simulink library "lindiCopter_lib"  (R2018b)
settings: Solver=VariableStepAuto  StartTime=0.0  StopTime=10.0  RelTol=1e-3
undefined symbols (not defined in the file or in its folder): lindi
libraries: filters_lib x5, indi_lib x4, cntrlPosNdi_lib x2, traj_lib x1, axes_transformation_lib x1, cntrlAttiRedIndi_lib x1
settings Model: Creator=Ybeyer  LastModifiedBy=yannic
settings SFSimCC: SimUseLocalCustomCode=off
settings RTWCC: RTWUseLocalCustomCode=off
settings CodeAppCC: StateflowObjectComments=on

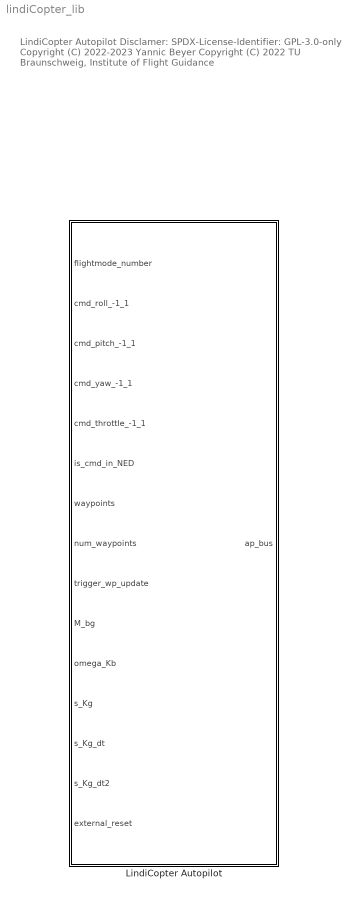
== system lindiCopter_lib ==
  note: LindiCopter Autopilot
      |
      | Disclamer:
      | SPDX-License-Identifier: GPL-3.0-only
      |
      | Copyright (C) 2022-2023 Yannic Beyer
      | Copyright (C) 2022 TU Braunschweig, Institute of Flight Guidance
  LindiCopter Autopilot : Subsystem  mask{ap=lindi}
      mask prompts: ap "LinidCopter parameters struct, see lindiCopter_params_default"
      mask init:
      | lindiCopterStateLogicBus();
      mask Help: web('hhttps://github.com/iff-gsc/LADAC/tree/main/control/autopilots/LindiCopter/README.md','-browser')
      mask DialogControl DescGroupVar Prompt: LindiCopter Autopilot
      mask DialogControl Control4 Prompt: The documentation of this block can be found here:
      mask DialogControl Control5 Prompt: README
      mask DialogControl Control5 Callback: web('https://github.com/iff-gsc/LADAC/blob/main/control/autopilots/LindiCopter/README.md','-browser')

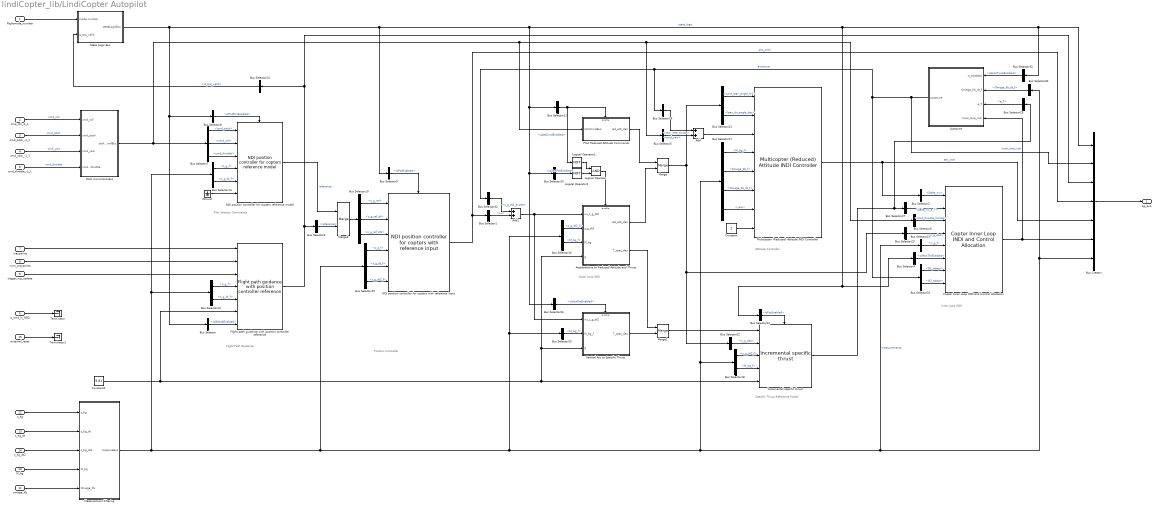
== system lindiCopter_lib/LindiCopter Autopilot ==
  note: Position Controller
  note: Flight Path Guidance
  note: Pilot Velocity Commands
  note: Outer Loop INDI
  note: Specific Thrust
      | Reference Model
  note: Attitude Controller
  note: Inner Loop INDI
  flightmode_number : Inport  SampleTime=ap.ts
  cmd_roll_-1_1 : Inport  Port=2  SampleTime=ap.ts
  cmd_pitch_-1_1 : Inport  Port=3  SampleTime=ap.ts
  cmd_yaw_-1_1 : Inport  Port=4  SampleTime=ap.ts
  cmd_throttle_-1_1 : Inport  Port=5  SampleTime=ap.ts
  is_cmd_in_NED : Inport  Port=6  SampleTime=ap.ts
  waypoints : Inport  Port=7  SampleTime=ap.ts
  num_waypoints : Inport  Port=8  SampleTime=ap.ts
  trigger_wp_update : Inport  Port=9  SampleTime=ap.ts
  M_bg : Inport  Port=10  SampleTime=ap.ts
  omega_Kb : Inport  Port=11  SampleTime=ap.ts
  s_Kg : Inport  Port=12  SampleTime=ap.ts
  s_Kg_dt : Inport  Port=13  SampleTime=ap.ts
  s_Kg_dt2 : Inport  Port=14  SampleTime=ap.ts
  external_reset : Inport  Port=15  SampleTime=ap.ts
  Accelerations to Reduced Attitude and Thrust : Subsystem
  Add : Sum
  Add1 : Sum
  Autotune : Subsystem
  Bus Creator : BusCreator  Inputs=7
  Bus Selector : BusSelector  OutputSignals=isGdnceEnabled
  Bus Selector1 : BusSelector  OutputSignals=pseudo_control.nu
  Bus Selector10 : BusSelector  OutputSignals=s_g_ref,s_g_ref_dt,s_g_ref_dt2
  Bus Selector11 : BusSelector  OutputSignals=isAttiCmdEnabled
  Bus Selector12 : BusSelector  OutputSignals=isPscEnabled
  Bus Selector13 : BusSelector  OutputSignals=s_g_f,s_g_dt_f
  Bus Selector14 : BusSelector  OutputSignals=s_g_f,s_g_dt_f
  Bus Selector15 : BusSelector  OutputSignals=s_g_f,s_g_dt_f,s_g_dt2_f
  Bus Selector16 : BusSelector  OutputSignals=s_g_dt2_f,M_bg_f
  Bus Selector17 : BusSelector  OutputSignals=M_bg_f,Omega_Kb_f,Omega_Kb_dt_f,yaw
  Bus Selector18 : BusSelector  OutputSignals=s_g_dt2_f,M_bg_f
  Bus Selector19 : BusSelector  OutputSignals=n_g_f
  Bus Selector2 : BusSelector  OutputSignals=pseudo_control.Delta_ny
  Bus Selector20 : BusSelector  OutputSignals=isVertPscEnabled
  Bus Selector21 : BusSelector  OutputSignals=cmd_lean_angle_0-1,lean_dir_angle_des
  Bus Selector22 : BusSelector  OutputSignals=n_g_des
  Bus Selector23 : BusSelector  OutputSignals=n_g_des
  Bus Selector24 : BusSelector  OutputSignals=is_traj_valid
  Bus Selector25 : BusSelector  OutputSignals=M_bg_f
  Bus Selector26 : BusSelector  OutputSignals=isVertPscEnabled
  Bus Selector27 : BusSelector  OutputSignals=Delta_nu_a_T
  Bus Selector28 : BusSelector  OutputSignals=excite.yaw_rate_excite
  Bus Selector29 : BusSelector  OutputSignals=a_T
  Bus Selector3 : BusSelector  OutputSignals=reference
  Bus Selector30 : BusSelector  OutputSignals=Omega_Kb_dt_f
  Bus Selector31 : BusSelector  OutputSignals=G1_adapt,G2_adapt
  Bus Selector32 : BusSelector  OutputSignals=excite.s_g_dt2_excite
  Bus Selector33 : BusSelector  OutputSignals=isAutoTuneEnabled
  Bus Selector4 : BusSelector  OutputSignals=isManThrEnabled
  Bus Selector5 : BusSelector  OutputSignals=cmd_yaw
  Bus Selector6 : BusSelector  OutputSignals=cmd_throttle_limited
  Bus Selector7 : BusSelector  OutputSignals=cmd_pitch,cmd_roll,cmd_throttle
  Bus Selector8 : BusSelector  OutputSignals=isPosRmEnabled
  Bus Selector9 : BusSelector  OutputSignals=isPscEnabled
  Constant : Constant
  Constant2 : Constant  Value=9.81
  Copter Inner Loop INDI and Control Allocation : indi_lib/Copter Inner Loop INDI and Control Allocation  cep=ap.cep  ceb=ap.ceb  ca=ap.ca  mtc=ap.mtc  sflt=ap.sflt  ts=ap.ts  is_ce_extern=on
      settings: SourceProductName=LADAC
  Flight path guidance with position controller reference : traj_lib/Flight path guidance with position controller reference  traj_params=ap.traj  T_inner_loop=2./ap.atc.rm.leanfreq + ap.mtc + 2./ap.sflt.omega
      settings: SourceProductName=LADAC
  Ground : Ground
  Incremental specific thrust : indi_lib/Incremental specific thrust  leanfreq=ap.atc.rm.leanfreq  leandamp=ap.atc.rm.leandamp  is_enable_checked=on  states_when_enabling=held
      settings: SourceProductName=LADAC
  Logical Operator : Logic  AllPortsSameDT=off  OutDataTypeStr=boolean
  Logical Operator1 : Logic  Operator=NOT  AllPortsSameDT=off  OutDataTypeStr=boolean
  Logical Operator2 : Logic  Operator=NOT  AllPortsSameDT=off  OutDataTypeStr=boolean
  Measurement Filtering : Subsystem
  Merge : Merge
  Merge1 : Merge
  Merge3 : Merge
  Multicopter (Reduced) Attitude INDI Controller : cntrlAttiRedIndi_lib/Multicopter (Reduced) Attitude INDI Controller  atc=ap.atc  T=ap.mtc + 2./ap.sflt.omega
      settings: SourceProductName=LADAC
  NDI position controller for copters reference model : cntrlPosNdi_lib/NDI position controller for copters reference model  psc=ap.psc  is_enable_checked=on  states_when_enabling=reset
      settings: SourceProductName=LADAC
  NDI position controller for copters with reference input : cntrlPosNdi_lib/NDI position controller for copters with reference input  psc=ap.psc  T_inner_loop=2./ap.atc.rm.leanfreq + ap.mtc + 2./ap.sflt.omega  is_enable_checked=on  states_when_enabling=reset
      settings: SourceProductName=LADAC
  Pilot Reduced Attitude Commands : Subsystem
  State Logic Bus : Subsystem
  Stick Command Bus : Subsystem  mask{thr=ap.thr}
      mask prompts: thr "Throttle parameters"
      mask DialogControl DescGroupVar Prompt: Stick Commands
  Terminator : Terminator
  Terminator1 : Terminator
  Vertical Acc to Specific Thrust : Subsystem
  ap_bus : Outport  SampleTime=ap.ts
  wires:
  Bus Selector24/1 -> State Logic Bus/2(is_traj_valid)  "<is_traj_valid>"
  Add1/1 -> Vertical Acc to Specific Thrust/1(nu_z_g_dt2), Accelerations to Reduced Attitude and Thrust/1(nu_s_g_dt2)
  Bus Selector3/1 -> Merge3/2  "<reference>"
  Merge3/1 -> Bus Selector10/1
  Bus Selector20/1 -> Logical Operator2/1  "<isVertPscEnabled>"
  Bus Selector2/1 -> Copter Inner Loop INDI and Control Allocation/1  "<Delta_ny>"
  Copter Inner Loop INDI and Control Allocation/1 -> Autotune/4(inner_loop_indi), Bus Creator/6  "inner_loop_indi"
  Multicopter (Reduced) Attitude INDI Controller/1 -> Bus Selector2/1, Bus Creator/5  "atti_cntrl"
  is_cmd_in_NED/1 -> Terminator/1
  Bus Creator/1 -> ap_bus/1
  Bus Selector1/1 -> Add1/2  "<nu>"
  NDI position controller for copters with reference input/1 -> Bus Selector1/1, Bus Creator/4  "pos_cntrl"
  Constant/1 -> Multicopter (Reduced) Attitude INDI Controller/8
  Bus Selector10/3 -> NDI position controller for copters with reference input/3  "<s_g_ref_dt2>"
  Bus Selector10/2 -> NDI position controller for copters with reference input/2  "<s_g_ref_dt>"
  Bus Selector10/1 -> NDI position controller for copters with reference input/1  "<s_g_ref>"
  Constant2/1 -> Flight path guidance with position controller reference/6, Incremental specific thrust/5, Vertical Acc to Specific Thrust/3(g), Accelerations to Reduced Attitude and Thrust/4(g)
  NDI position controller for copters reference model/1 -> Merge3/1  "reference"
  flightmode_number/1 -> State Logic Bus/1(mode number)
  external_reset/1 -> Terminator1/1
  Merge1/1 -> Incremental specific thrust/1
  Incremental specific thrust/1 -> Bus Selector27/1, Bus Selector29/1
  omega_Kb/1 -> Measurement Filtering/5(Omega_Kb)
  M_bg/1 -> Measurement Filtering/4(M_bg)
  s_Kg_dt2/1 -> Measurement Filtering/3(s_Kg_dt2)
  s_Kg_dt/1 -> Measurement Filtering/2(s_Kg_dt)
  s_Kg/1 -> Measurement Filtering/1(s_Kg)
  State Logic Bus/1(stateLogicBus) -> Bus Selector8/1, Bus Selector/1, Bus Selector9/1, Bus Selector26/1, Bus Selector20/1, Bus Selector11/1, Bus Selector12/1, Bus Selector4/1, Bus Selector33/1, Bus Creator/1  "state_logic"
  Bus Selector4/1 -> Copter Inner Loop INDI and Control Allocation/6  "<isManThrEnabled>"
  Add/1 -> Multicopter (Reduced) Attitude INDI Controller/3
  Bus Selector6/1 -> Copter Inner Loop INDI and Control Allocation/3  "<cmd_throttle_limited>"
  Bus Selector7/3 -> NDI position controller for copters reference model/3  "<cmd_throttle>"
  Bus Selector7/1 -> NDI position controller for copters reference model/1  "<cmd_pitch>"
  Bus Selector7/2 -> NDI position controller for copters reference model/2  "<cmd_roll>"
  Flight path guidance with position controller reference/1 -> Bus Creator/3, Bus Selector24/1, Bus Selector3/1
  waypoints/1 -> Flight path guidance with position controller reference/1
  trigger_wp_update/1 -> Flight path guidance with position controller reference/3
  Bus Selector/1 -> Flight path guidance with position controller reference/7  "<isGdnceEnabled>"
  Bus Selector8/1 -> NDI position controller for copters reference model/Enable  "<isPosRmEnabled>"
  Bus Selector9/1 -> NDI position controller for copters with reference input/Enable  "<isPscEnabled>"
  Bus Selector11/1 -> Logical Operator1/1, Pilot Reduced Attitude Commands/Enable  "<isAttiCmdEnabled>"
  Bus Selector12/1 -> Incremental specific thrust/Enable  "<isPscEnabled>"
  Ground/1 -> NDI position controller for copters reference model/6
  Measurement Filtering/1(measureBus) -> Bus Selector15/1, Bus Selector16/1, Bus Selector25/1, Bus Selector19/1, Bus Selector30/1, Bus Creator/7, Bus Selector18/1, Bus Selector17/1, Bus Selector14/1, Bus Selector13/1  "measurements"
  Bus Selector13/1 -> Flight path guidance with position controller reference/4  "<s_g_f>"
  Bus Selector13/2 -> Flight path guidance with position controller reference/5  "<s_g_dt_f>"
  Bus Selector14/1 -> NDI position controller for copters reference model/4  "<s_g_f>"
  Bus Selector14/2 -> NDI position controller for copters reference model/5  "<s_g_dt_f>"
  Bus Selector15/1 -> NDI position controller for copters with reference input/4  "<s_g_f>"
  Bus Selector15/2 -> NDI position controller for copters with reference input/5  "<s_g_dt_f>"
  Bus Selector15/3 -> NDI position controller for copters with reference input/6  "<s_g_dt2_f>"
  Bus Selector16/1 -> Accelerations to Reduced Attitude and Thrust/2(s_g_dt2)  "<s_g_dt2_f>"
  Bus Selector16/2 -> Accelerations to Reduced Attitude and Thrust/3(M_bg)  "<M_bg_f>"
  Bus Selector17/1 -> Multicopter (Reduced) Attitude INDI Controller/4  "<M_bg_f>"
  Bus Selector17/2 -> Multicopter (Reduced) Attitude INDI Controller/5  "<Omega_Kb_f>"
  Bus Selector17/3 -> Multicopter (Reduced) Attitude INDI Controller/6  "<Omega_Kb_dt_f>"
  Bus Selector18/1 -> Incremental specific thrust/3  "<s_g_dt2_f>"
  Bus Selector18/2 -> Incremental specific thrust/4  "<M_bg_f>"
  Bus Selector22/1 -> Incremental specific thrust/2  "<n_g_des>"
  Bus Selector19/1 -> Copter Inner Loop INDI and Control Allocation/5  "<n_g_f>"
  Bus Selector17/4 -> Multicopter (Reduced) Attitude INDI Controller/7  "<yaw>"
  Stick Command Bus/1(stickCmdBus) -> Pilot Reduced Attitude Commands/1(stickCmdBus), Bus Selector6/1, Bus Selector5/1, Bus Selector7/1
  cmd_roll_-1_1/1 -> Stick Command Bus/1(cmd_roll)  "cmd_roll"
  cmd_pitch_-1_1/1 -> Stick Command Bus/2(cmd_pitch)  "cmd_pitch"
  cmd_yaw_-1_1/1 -> Stick Command Bus/3(cmd_yaw)  "cmd_yaw"
  cmd_throttle_-1_1/1 -> Stick Command Bus/4(cmd_throttle)  "cmd_throttle"
  Bus Selector21/1 -> Multicopter (Reduced) Attitude INDI Controller/1  "<cmd_lean_angle_0-1>"
  Bus Selector21/2 -> Multicopter (Reduced) Attitude INDI Controller/2  "<lean_dir_angle_des>"
  Merge/1 -> Bus Selector21/1, Bus Selector22/1, Bus Selector23/1
  Pilot Reduced Attitude Commands/1(red_atti_des) -> Merge/1
  Bus Selector23/1 -> Copter Inner Loop INDI and Control Allocation/4  "<n_g_des>"
  Accelerations to Reduced Attitude and Thrust/1(red_atti_des) -> Merge/2
  Accelerations to Reduced Attitude and Thrust/2(T_spec_des) -> Merge1/1
  Vertical Acc to Specific Thrust/1(T_spec_des) -> Merge1/2
  Bus Selector25/1 -> Vertical Acc to Specific Thrust/2(M_bg_f)  "<M_bg_f>"
  Bus Selector26/1 -> Vertical Acc to Specific Thrust/Enable  "<isVertPscEnabled>"
  Logical Operator1/1 -> Logical Operator/1
  Logical Operator2/1 -> Logical Operator/2
  Logical Operator/1 -> Accelerations to Reduced Attitude and Thrust/Enable
  Bus Selector27/1 -> Copter Inner Loop INDI and Control Allocation/2  "<Delta_nu_a_T>"
  Bus Selector31/2 -> Copter Inner Loop INDI and Control Allocation/8  "<G2_adapt>"
  Bus Selector31/1 -> Copter Inner Loop INDI and Control Allocation/7  "<G1_adapt>"
  Bus Selector30/1 -> Autotune/2(Omega_Kb_dt_f)  "<Omega_Kb_dt_f>"
  Bus Selector29/1 -> Autotune/3(a_T)  "<a_T>"
  Autotune/1(autotune) -> Bus Creator/2, Bus Selector31/1, Bus Selector28/1, Bus Selector32/1  "autotune"
  Bus Selector28/1 -> Add/1  "<yaw_rate_excite>"
  Bus Selector32/1 -> Add1/1  "<s_g_dt2_excite>"
  Bus Selector33/1 -> Autotune/1(is_enabled)  "<isAutoTuneEnabled>"
  Bus Selector5/1 -> Add/2  "<cmd_yaw>"
  num_waypoints/1 -> Flight path guidance with position controller reference/2

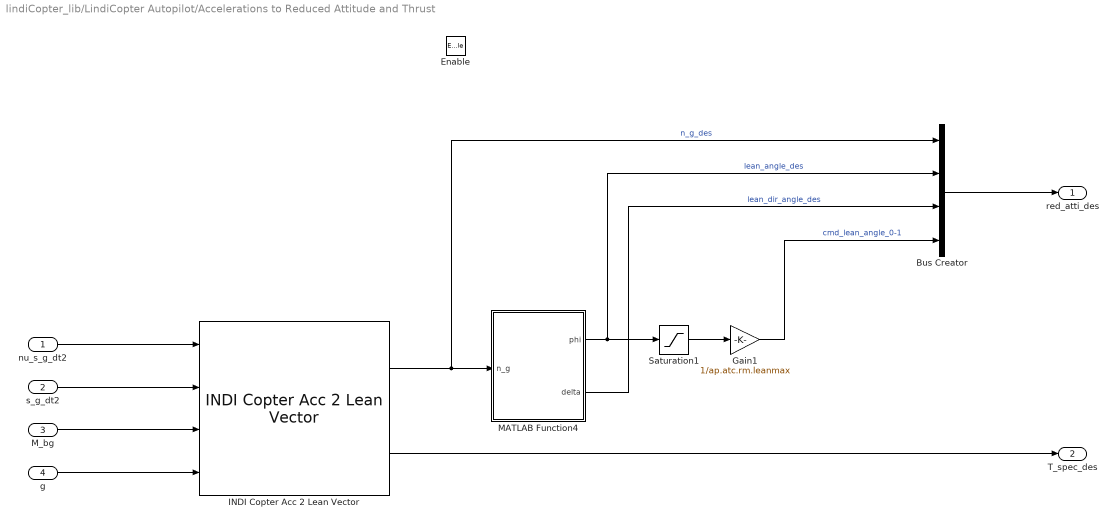
== system lindiCopter_lib/LindiCopter Autopilot/Accelerations to Reduced Attitude and Thrust ==
  nu_s_g_dt2 : Inport
  s_g_dt2 : Inport  Port=2
  M_bg : Inport  Port=3
  g : Inport  Port=4
  Enable : EnablePort
  Bus Creator : BusCreator  Inputs=4
  Gain1 : Gain  Gain=1/ap.atc.rm.leanmax
  INDI Copter Acc 2 Lean Vector : indi_lib/INDI Copter Acc 2 Lean Vector  SystemSampleTime=-1
      settings: SourceProductName=LADAC
  MATLAB Function4 : MATLAB Function  TreatAsAtomicUnit=on
  Saturation1 : Saturate  UpperLimit=ap.atc.rm.leanmax  LowerLimit=0
  red_atti_des : Outport
  T_spec_des : Outport  Port=2
  wires:
  MATLAB Function4/2(delta) -> Bus Creator/3  "lean_dir_angle_des"
  Gain1/1 -> Bus Creator/4  "cmd_lean_angle_0-1"
  nu_s_g_dt2/1 -> INDI Copter Acc 2 Lean Vector/1
  Saturation1/1 -> Gain1/1
  MATLAB Function4/1(phi) -> Bus Creator/2, Saturation1/1  "lean_angle_des"
  g/1 -> INDI Copter Acc 2 Lean Vector/4
  s_g_dt2/1 -> INDI Copter Acc 2 Lean Vector/2
  M_bg/1 -> INDI Copter Acc 2 Lean Vector/3
  INDI Copter Acc 2 Lean Vector/1 -> Bus Creator/1, MATLAB Function4/1(n_g)  "n_g_des"
  INDI Copter Acc 2 Lean Vector/2 -> T_spec_des/1
  Bus Creator/1 -> red_atti_des/1

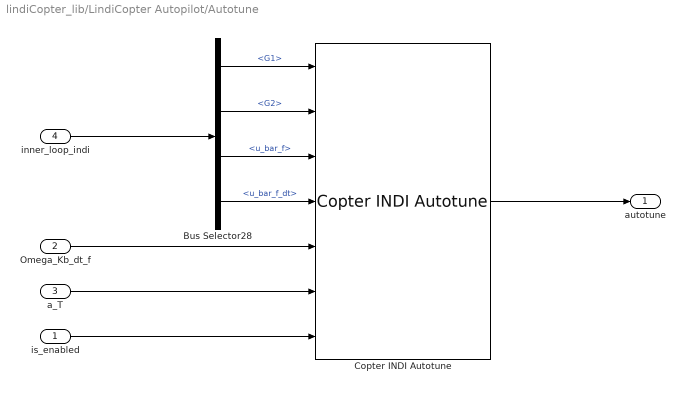
== system lindiCopter_lib/LindiCopter Autopilot/Autotune ==
  is_enabled : Inport
  Omega_Kb_dt_f : Inport  Port=2
  a_T : Inport  Port=3
  inner_loop_indi : Inport  Port=4
  Bus Selector28 : BusSelector  OutputSignals=G1,G2,u_bar_f,u_bar_f_dt
  Copter INDI Autotune : indi_lib/Copter INDI Autotune  rm_atc=ap.atc.rm  mtc=ap.mtc  sflt_omega=ap.sflt.omega  ts=ap.ts
      settings: SourceProductName=LADAC
  autotune : Outport
  wires:
  is_enabled/1 -> Copter INDI Autotune/7
  Bus Selector28/4 -> Copter INDI Autotune/4  "<u_bar_f_dt>"
  Bus Selector28/2 -> Copter INDI Autotune/2  "<G2>"
  inner_loop_indi/1 -> Bus Selector28/1
  Bus Selector28/1 -> Copter INDI Autotune/1  "<G1>"
  Bus Selector28/3 -> Copter INDI Autotune/3  "<u_bar_f>"
  Copter INDI Autotune/1 -> autotune/1
  a_T/1 -> Copter INDI Autotune/6
  Omega_Kb_dt_f/1 -> Copter INDI Autotune/5

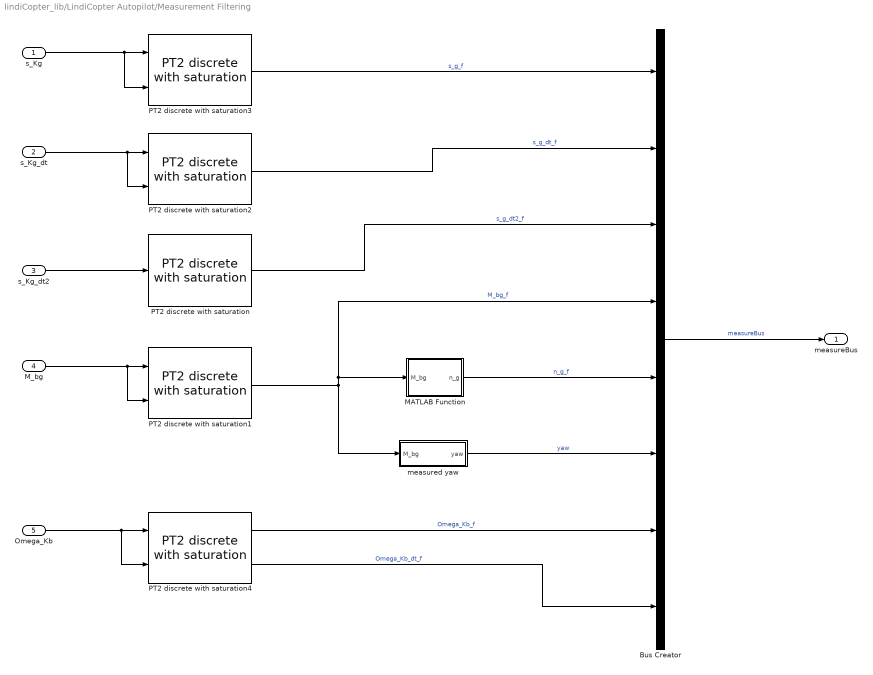
== system lindiCopter_lib/LindiCopter Autopilot/Measurement Filtering ==
  s_Kg : Inport
  s_Kg_dt : Inport  Port=2
  s_Kg_dt2 : Inport  Port=3
  M_bg : Inport  Port=4
  Omega_Kb : Inport  Port=5
  Bus Creator : BusCreator  Inputs=8
  MATLAB Function : MATLAB Function  TreatAsAtomicUnit=on
  PT2 discrete with saturation : filters_lib/PT2 discrete with saturation  param_src=internal  omega=ap.sflt.omega  d=ap.sflt.D  x_dt2_max=inf  x_dt2_min=-inf  x_dt_max=inf  x_dt_min=-inf  x_max=inf  x_min=-inf  y_0_src=internal  x_init=0  y_dt_0_src=internal  x_dt_init=0  is_y_dt_checked=off  is_y_dt2_checked=off
      settings: SourceProductName=LADAC
  PT2 discrete with saturation1 : filters_lib/PT2 discrete with saturation  param_src=internal  omega=ap.sflt.omega  d=ap.sflt.D  x_dt2_max=inf  x_dt2_min=-inf  x_dt_max=inf  x_dt_min=-inf  x_max=inf  x_min=-inf  y_0_src=external  x_init=0  y_dt_0_src=internal  x_dt_init=0  is_y_dt_checked=off  is_y_dt2_checked=off
      settings: SourceProductName=LADAC
  PT2 discrete with saturation2 : filters_lib/PT2 discrete with saturation  param_src=internal  omega=ap.sflt.omega  d=ap.sflt.D  x_dt2_max=inf  x_dt2_min=-inf  x_dt_max=inf  x_dt_min=-inf  x_max=inf  x_min=-inf  y_0_src=external  x_init=0  y_dt_0_src=internal  x_dt_init=0  is_y_dt_checked=off  is_y_dt2_checked=off
      settings: SourceProductName=LADAC
  PT2 discrete with saturation3 : filters_lib/PT2 discrete with saturation  param_src=internal  omega=ap.sflt.omega  d=ap.sflt.D  x_dt2_max=inf  x_dt2_min=-inf  x_dt_max=inf  x_dt_min=-inf  x_max=inf  x_min=-inf  y_0_src=external  x_init=0  y_dt_0_src=internal  x_dt_init=0  is_y_dt_checked=off  is_y_dt2_checked=off
      settings: SourceProductName=LADAC
  PT2 discrete with saturation4 : filters_lib/PT2 discrete with saturation  param_src=internal  omega=ap.sflt.omega  d=ap.sflt.D  x_dt2_max=inf  x_dt2_min=-inf  x_dt_max=inf  x_dt_min=-inf  x_max=inf  x_min=-inf  y_0_src=external  x_init=0  y_dt_0_src=internal  x_dt_init=0  is_y_dt_checked=on  is_y_dt2_checked=off
      settings: SourceProductName=LADAC
  measured yaw : Subsystem
  measureBus : Outport
  wires:
  PT2 discrete with saturation4/2 -> Bus Creator/8  "Omega_Kb_dt_f"
  Omega_Kb/1 -> PT2 discrete with saturation4/2, PT2 discrete with saturation4/1
  PT2 discrete with saturation4/1 -> Bus Creator/7  "Omega_Kb_f"
  M_bg/1 -> PT2 discrete with saturation1/1, PT2 discrete with saturation1/2
  PT2 discrete with saturation1/1 -> MATLAB Function/1(M_bg), Bus Creator/4, measured yaw/1(M_bg)  "M_bg_f"
  PT2 discrete with saturation/1 -> Bus Creator/3  "s_g_dt2_f"
  s_Kg_dt2/1 -> PT2 discrete with saturation/1
  PT2 discrete with saturation2/1 -> Bus Creator/2  "s_g_dt_f"
  s_Kg_dt/1 -> PT2 discrete with saturation2/1, PT2 discrete with saturation2/2
  PT2 discrete with saturation3/1 -> Bus Creator/1  "s_g_f"
  s_Kg/1 -> PT2 discrete with saturation3/2, PT2 discrete with saturation3/1
  MATLAB Function/1(n_g) -> Bus Creator/5  "n_g_f"
  Bus Creator/1 -> measureBus/1  "measureBus"
  measured yaw/1(yaw) -> Bus Creator/6  "yaw"

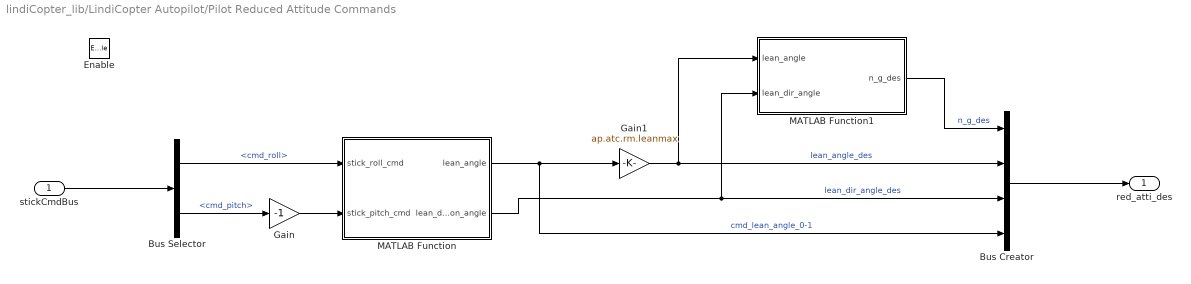
== system lindiCopter_lib/LindiCopter Autopilot/Pilot Reduced Attitude Commands ==
  stickCmdBus : Inport
  Enable : EnablePort
  Bus Creator : BusCreator  Inputs=4
  Bus Selector : BusSelector  OutputSignals=cmd_roll,cmd_pitch
  Gain : Gain  Gain=-1
  Gain1 : Gain  Gain=ap.atc.rm.leanmax
  MATLAB Function : MATLAB Function  TreatAsAtomicUnit=on
  MATLAB Function1 : MATLAB Function  TreatAsAtomicUnit=on
  red_atti_des : Outport
  wires:
  Gain/1 -> MATLAB Function/2(stick_pitch_cmd)
  Bus Selector/1 -> MATLAB Function/1(stick_roll_cmd)  "<cmd_roll>"
  Bus Selector/2 -> Gain/1  "<cmd_pitch>"
  stickCmdBus/1 -> Bus Selector/1
  MATLAB Function/2(lean_direction_angle) -> MATLAB Function1/2(lean_dir_angle), Bus Creator/3  "lean_dir_angle_des"
  Gain1/1 -> Bus Creator/2, MATLAB Function1/1(lean_angle)  "lean_angle_des"
  MATLAB Function1/1(n_g_des) -> Bus Creator/1  "n_g_des"
  Bus Creator/1 -> red_atti_des/1
  MATLAB Function/1(lean_angle) -> Bus Creator/4, Gain1/1  "cmd_lean_angle_0-1"

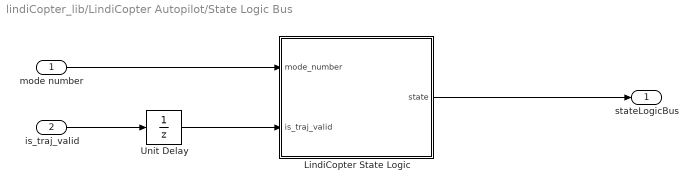
== system lindiCopter_lib/LindiCopter Autopilot/State Logic Bus ==
  mode number : Inport
  is_traj_valid : Inport  Port=2
  LindiCopter State Logic : MATLAB Function  TreatAsAtomicUnit=on
  Unit Delay : UnitDelay  SampleTime=-1
  stateLogicBus : Outport
  wires:
  is_traj_valid/1 -> Unit Delay/1
  mode number/1 -> LindiCopter State Logic/1(mode_number)
  LindiCopter State Logic/1(state) -> stateLogicBus/1
  Unit Delay/1 -> LindiCopter State Logic/2(is_traj_valid)

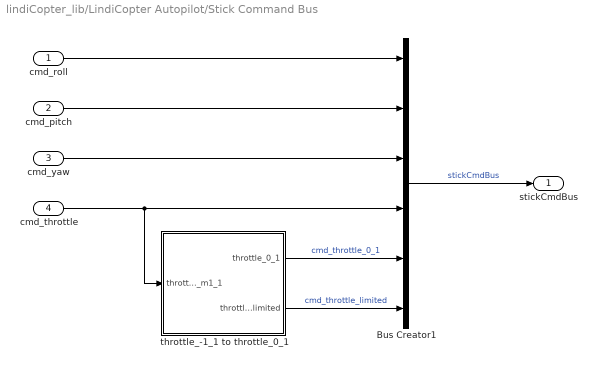
== system lindiCopter_lib/LindiCopter Autopilot/Stick Command Bus ==
  cmd_roll : Inport
  cmd_pitch : Inport  Port=2
  cmd_yaw : Inport  Port=3
  cmd_throttle : Inport  Port=4
  Bus Creator1 : BusCreator  Inputs=6
  throttle_-1_1 to throttle_0_1 : MATLAB Function  TreatAsAtomicUnit=on
  stickCmdBus : Outport
  wires:
  cmd_roll/1 -> Bus Creator1/1
  throttle_-1_1 to throttle_0_1/1(throttle_0_1) -> Bus Creator1/5  "cmd_throttle_0_1"
  Bus Creator1/1 -> stickCmdBus/1  "stickCmdBus"
  cmd_yaw/1 -> Bus Creator1/3
  cmd_throttle/1 -> throttle_-1_1 to throttle_0_1/1(throttle_m1_1), Bus Creator1/4
  cmd_pitch/1 -> Bus Creator1/2
  throttle_-1_1 to throttle_0_1/2(throttle_limited) -> Bus Creator1/6  "cmd_throttle_limited"

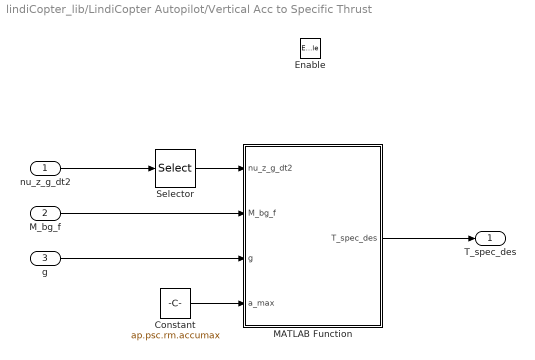
== system lindiCopter_lib/LindiCopter Autopilot/Vertical Acc to Specific Thrust ==
  nu_z_g_dt2 : Inport
  M_bg_f : Inport  Port=2
  g : Inport  Port=3
  Enable : EnablePort
  Constant : Constant  Value=ap.psc.rm.accumax
  MATLAB Function : MATLAB Function  TreatAsAtomicUnit=on
  Selector : Selector  InputPortWidth=3  IndexOptions=Index vector (dialog)  Indices=3  OutputSizes=1
  T_spec_des : Outport
  wires:
  Constant/1 -> MATLAB Function/4(a_max)
  Selector/1 -> MATLAB Function/1(nu_z_g_dt2)
  nu_z_g_dt2/1 -> Selector/1
  M_bg_f/1 -> MATLAB Function/2(M_bg_f)
  MATLAB Function/1(T_spec_des) -> T_spec_des/1
  g/1 -> MATLAB Function/3(g)

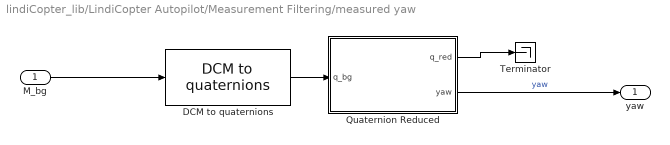
== system lindiCopter_lib/LindiCopter Autopilot/Measurement Filtering/measured yaw ==
  M_bg : Inport
  DCM to quaternions : axes_transformation_lib/DCM to quaternions  SystemSampleTime=-1
      settings: SourceProductName=LADAC
  Quaternion Reduced : MATLAB Function  TreatAsAtomicUnit=on
  Terminator : Terminator
  yaw : Outport
  wires:
  DCM to quaternions/1 -> Quaternion Reduced/1(q_bg)
  Quaternion Reduced/1(q_red) -> Terminator/1
  Quaternion Reduced/2(yaw) -> yaw/1  "yaw"
  M_bg/1 -> DCM to quaternions/1

== matlab function lindiCopter_lib/LindiCopter Autopilot/Measurement Filtering/MATLAB Function ==
  data: M_bg input; n_g output
function n_g = dcm2LeanVector( M_bg )
n_g = dcm2LeanVector( M_bg );
end

== matlab function lindiCopter_lib/LindiCopter Autopilot/Pilot Reduced Attitude Commands/MATLAB Function ==
  data: stick_roll_cmd input; lean_angle output; stick_pitch_cmd input; lean_direction_angle output
function [lean_angle,lean_direction_angle] = fcn(stick_roll_cmd,stick_pitch_cmd)

lean_angle = sqrt( stick_roll_cmd^2 + stick_pitch_cmd^2 );
lean_direction_angle = atan2(stick_roll_cmd,-stick_pitch_cmd);

end

== matlab function lindiCopter_lib/LindiCopter Autopilot/Pilot Reduced Attitude Commands/MATLAB Function1 ==
  data: lean_angle input; n_g_des output; lean_dir_angle input
function n_g_des = fcn(lean_angle,lean_dir_angle)

n_g_des = leanAngles2leanVector([lean_angle,lean_dir_angle]);

end

== matlab function lindiCopter_lib/LindiCopter Autopilot/State Logic Bus/LindiCopter State Logic ==
  data: mode_number input; state output Bus: lindiStateLogicBus; is_traj_valid input
function state = lindiCopterStateLogic(mode_number, is_traj_valid)
state = lindiCopterStateLogic(mode_number,is_traj_valid);
end

== matlab function lindiCopter_lib/LindiCopter Autopilot/Accelerations to Reduced Attitude and Thrust/MATLAB Function4 ==
  data: n_g input; phi output; delta output
function [phi,delta] = leanVector2LeanAngles(n_g)
[phi,delta] = leanVector2LeanAngles(n_g);
end

== matlab function lindiCopter_lib/LindiCopter Autopilot/Vertical Acc to Specific Thrust/MATLAB Function ==
  data: nu_z_g_dt2 input; M_bg_f input; T_spec_des output; g input; a_max input
function T_spec_des = fcn(nu_z_g_dt2,M_bg_f,g,a_max)
den = M_bg_f(3,3);
T_spec_des = zeros(1,1,superiorfloat(nu_z_g_dt2(1)));
if den < g/a_max
    T_spec_des(:) = 0;
else
    T_spec_des(:) = divideFinite(-nu_z_g_dt2+g,den);
end
end

== matlab function lindiCopter_lib/LindiCopter Autopilot/Stick Command Bus/throttle_-1_1 to throttle_0_1 ==
  data: throttle_m1_1 input; throttle_0_1 output; thr parameter; throttle_limited output
function [throttle_0_1,throttle_limited] = fcn(throttle_m1_1,thr)
throttle_0_1 = max(0,min(1,0.5+0.5*throttle_m1_1));
throttle_limited = thr.min + (thr.max-thr.min)*throttle_0_1;
end

== matlab function lindiCopter_lib/LindiCopter Autopilot/Measurement Filtering/measured yaw/Quaternion Reduced ==
  data: q_bg input; q_red output; yaw output
function [q_red,yaw] = fcn(q_bg)
[q_red,yaw] = quatReduced(q_bg);
end
